simulink model "ex_04_1_sim"  (R2024b)
settings: Solver=VariableStepAuto  StartTime=0.0  StopTime=10.0  RelTol=1e-3
undefined symbols (not defined in the file or in its folder): A, A_v, B, B_v, c, C, C_v, D, D_v, k_x, kyita1, kyita2, r, v_start, w
settings Model: Creator=54238  LastModifiedBy=54238

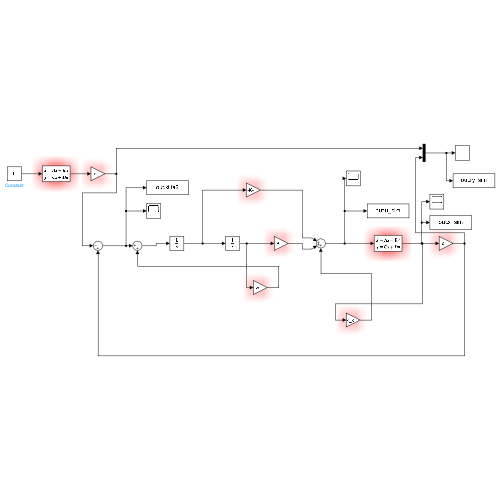
[thumbnail: Simulink's stored preview of the top-level diagram]
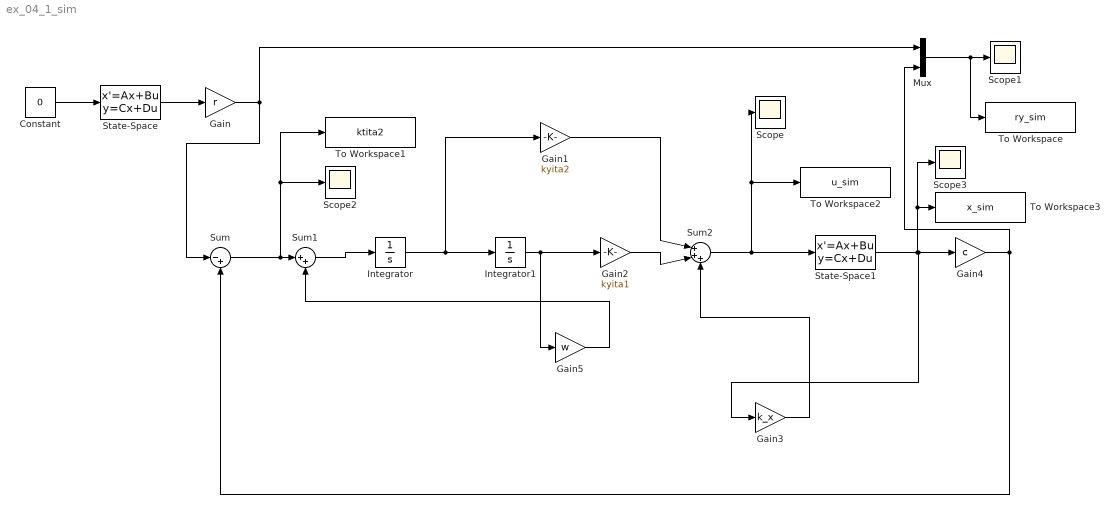
== system ex_04_1_sim ==
  Constant : Constant  Value=0
  Gain : Gain  Gain=r
  Gain1 : Gain  Gain=kyita2
  Gain2 : Gain  Gain=kyita1
  Gain3 : Gain  Gain=k_x
  Gain4 : Gain  Gain=c
  Gain5 : Gain  Gain=w
  Integrator : Integrator
  Integrator1 : Integrator
  Mux : Mux  Inputs=2
  Scope{,1..3} (4 alike) : Scope
  State-Space : StateSpace  A=A_v  B=B_v  C=C_v  D=D_v  InitialCondition=v_start
  State-Space1 : StateSpace  A=A  B=B  C=C  D=D  InitialCondition=0
  Sum : Sum  Inputs=|-+
  Sum1 : Sum  Inputs=|++
  Sum2 : Sum  Inputs=|+++
  To Workspace : ToWorkspace  VariableName=ry_sim  SaveFormat=Timeseries  SampleTime=-1
  To Workspace1 : ToWorkspace  VariableName=ktita2  SaveFormat=Timeseries  SampleTime=-1
  To Workspace2 : ToWorkspace  VariableName=u_sim  SaveFormat=Timeseries  SampleTime=-1
  To Workspace3 : ToWorkspace  VariableName=x_sim  SaveFormat=Timeseries  SampleTime=-1
  wires:
  State-Space/1 -> Gain/1
  Gain/1 -> Mux/1, Sum/1
  Mux/1 -> To Workspace/1, Scope1/1
  Sum/1 -> To Workspace1/1, Scope2/1, Sum1/1
  Sum1/1 -> Integrator/1
  Integrator/1 -> Gain1/1, Integrator1/1
  Integrator1/1 -> Gain5/1, Gain2/1
  Gain5/1 -> Sum1/2
  Gain1/1 -> Sum2/1
  Gain2/1 -> Sum2/2
  Sum2/1 -> To Workspace2/1, Scope/1, State-Space1/1
  State-Space1/1 -> Scope3/1, To Workspace3/1, Gain3/1, Gain4/1
  Gain4/1 -> Sum/2, Mux/2
  Gain3/1 -> Sum2/3
  Constant/1 -> State-Space/1
